simulink model "simulink_controller"  (R2026a)
settings: Solver=VariableStepAuto
libraries: cstblocks_lti x3
settings Model: Creator=lilylz2  LastModifiedBy=lilylz2

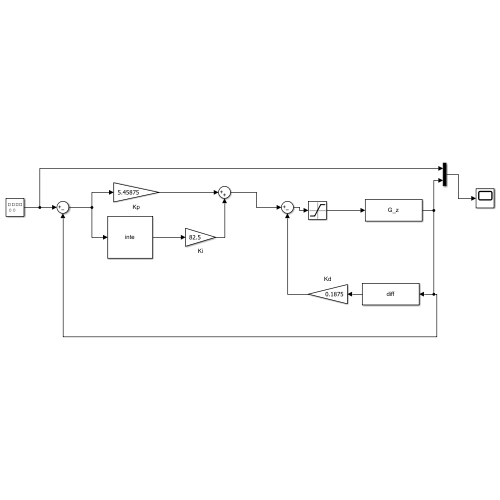
[thumbnail: Simulink's stored preview of the top-level diagram]
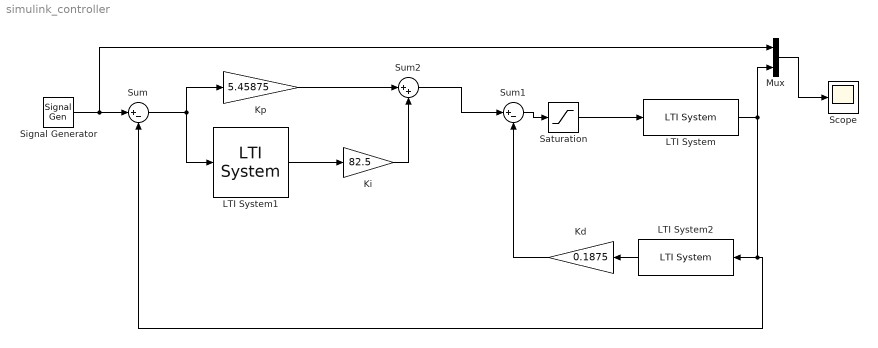
== system simulink_controller ==
  Kd : Gain  Gain=0.1875
  Ki : Gain  Gain=82.5
  Kp : Gain  Gain=5.45875
  LTI System : cstblocks_lti/LTI System  sys=G_z  IC=[]  PadeOrder=0
      settings: LibrarySourceBlock=cstblocks/LTI System
  LTI System1 : cstblocks_lti/LTI System  sys=inte  IC=[]  PadeOrder=0
      settings: LibrarySourceBlock=cstblocks/LTI System
  LTI System2 : cstblocks_lti/LTI System  sys=diff  IC=[]  PadeOrder=0
      settings: LibrarySourceBlock=cstblocks/LTI System
  Mux : Mux  Inputs=2
  Saturation : Saturate  UpperLimit=10  LowerLimit=-10
  Scope : Scope
      settings: ActiveDisplayYMinimum=-1.0275987093114207  ActiveDisplayYMaximum=1.0244350778207449
  Signal Generator : SignalGenerator  WaveForm=square  Frequency=0.25
  Sum : Sum  Inputs=|+-
  Sum1 : Sum  Inputs=|+-
  Sum2 : Sum  Inputs=|++
  wires:
  Sum/1 -> LTI System1/1, Kp/1
  LTI System1/1 -> Ki/1
  Ki/1 -> Sum2/2
  Kp/1 -> Sum2/1
  Sum2/1 -> Sum1/1
  Sum1/1 -> Saturation/1
  Saturation/1 -> LTI System/1
  LTI System/1 -> Sum/2, LTI System2/1, Mux/2
  Kd/1 -> Sum1/2
  LTI System2/1 -> Kd/1
  Signal Generator/1 -> Mux/1, Sum/1
  Mux/1 -> Scope/1
